simulink model "generic_src"  (Simulink 10.3)
settings: Solver=ode45  StartTime=0.0  StopTime=inf  RelTol=1e-3  EnableMultiTasking=on
undefined symbols (not defined in the file or in its folder): Area_Front, Area_Rear, ay_max_off, ay_max_on, ay_per_mu_max_off, ay_per_mu_max_on, Brake_ratio, brake_valve_ctrl_kP, cat1mode1_higher, cat1mode1_lower, cat1mode2_higher, cat1mode2_lower, cat1mode3_higher, cat1mode3_lower, cat2mode1_higher, cat2mode1_lower, cat2mode2_higher, cat2mode2_lower, cat2mode3_higher, cat2mode3_lower, delta_vel, diff_lock_fac, diff_lock_off, diff_lock_on, ESP_ctrl_kD, ESP_ctrl_kI, ESP_ctrl_kP, ESP_ctrl_restore_kI, ESP_min_throttle_fac, f_ax, f_slip, g, higherlimit_highvel, higherlimit_lowvel, highervel_fac, highervelocity_fac, InitialConditionForIntegrator, limit_acc, limit_selectlow, limit_starting, limit_vdiff, locktime_throttle, lowerlimit_highvel, lowerlimit_lowvel, lowervel_fac, lowervelocity_fac, min_throttle, MPS2KMPH, MSR_ctrl_kD, MSR_ctrl_kI, MSR_ctrl_kP, MSR_min_throttle_fac, PID_kP_sideslip, PID_kP_yawrate, RADpS2RpM, rBrake, RpM2RADpS, SH_SL_switch, sideslip_vel_corr, sidesplip_deviation_max ... (+35)
libraries: CarMaker4SL x136, simulink x55, simulink_extras x6
(part 7 of 9)

== system generic_src/CarMaker/IPG Vehicle/Brake/HydBrakeCU Example/ESP Controller/ESP General System/Signal Handling ==
  ESP In : Inport
  Vehicle Params : Inport  Port=2
  " " : simulink_extras/Transformations/Degrees to Radians
  "  " : simulink_extras/Transformations/Degrees to Radians
  "   " : Gain  Gain=RpM2RADpS
  "     " : Gain  Gain=RpM2RADpS
  "      " : Gain  Gain=RpM2RADpS
  Bus Creator : BusCreator  Inputs=4
  Bus Creator1 : BusCreator  Inputs=4
  Bus Creator2 : BusCreator  Inputs=6
  Bus Creator3 : BusCreator  Inputs=2
  Bus Creator4 : BusCreator  Inputs=2
  Bus Creator5 : BusCreator  Inputs=1
  Bus Creator6 : BusCreator  Inputs=3
  Bus Selector1 : BusSelector  OutputSignals=WheelSpd FL [rpm],WheelSpd FR [rpm],WheelSpd RL [rpm],WheelSpd RR [rpm],Master Cylinder Pressure [bar],Throttle Valve Position,Sensor Longitudinal acceleration [g],Engine Speed [rpm],GearState [-],Torque Converter Speed [rpm],Sensor YawRate [degs],Steering Wheel Angle [deg],Sensor Lateral acceleration [g],Cylinder Pressure FL [bar],Cylinder Pressure FR [bar],Cylinder Pressure RL [bar],Cylinder Pressure RR [bar],Engine crankshaft output torque [Nm],Park Brake Position,Brake Pedal Position
  Bus Selector2 : BusSelector  OutputSignals=SteeringGeometry
  Bus Selector3 : BusSelector  OutputSignals=SteerWheelAng_In,SteerAng_Out
  Gain2 : Gain  Gain=g  SaturateOnIntegerOverflow=on  OutDataTypeStr=Inherit: Same as input  ParamDataTypeStr=Inherit: Same as input
  Gain7 : Gain  Gain=g  SaturateOnIntegerOverflow=on  OutDataTypeStr=Inherit: Same as input  ParamDataTypeStr=Inherit: Same as input
  Lookup Table Dynamic : simulink/Lookup Tables/Lookup Table Dynamic  LookUpMeth=Interpolation-Use End Values  OutDataType=fixdt('double')  OutScaling=[]  OutputDataTypeScalingMode=Specify via dialog  OutDataTypeStr=fixdt('double')  DoSatur=off
  Termiator : Terminator
  Terminator1 : Terminator
  Terminator2 : Terminator
  Terminator4 : Terminator
  rpmin2rad/s : Gain  Gain=RpM2RADpS
  Signal Bus Master Controller : Outport  VectorParamsAs1DForOutWhenUnconnected=off
  Signal Bus ESP : Outport  Port=2  VectorParamsAs1DForOutWhenUnconnected=off
  Signal Bus ASR : Outport  Port=3  VectorParamsAs1DForOutWhenUnconnected=off
  Signal Bus ABS : Outport  Port=4  VectorParamsAs1DForOutWhenUnconnected=off
  Signal Bus HSA : Outport  Port=5  VectorParamsAs1DForOutWhenUnconnected=off
  wires:
  "  "/1 -> Lookup Table Dynamic/1
  rpmin2rad/s/1 -> Bus Creator/1  "WheelSpd_FL"
  Bus Selector1/1 -> rpmin2rad/s/1  "<WheelSpd FL [rpm]>"
  Bus Selector1/2 -> "   "/1  "<WheelSpd FR [rpm]>"
  Bus Selector1/3 -> "     "/1  "<WheelSpd RL [rpm]>"
  Bus Selector1/4 -> "      "/1  "<WheelSpd RR [rpm]>"
  Bus Selector1/7 -> Gain7/1  "<Sensor Longitudinal acceleration [g]>"
  Bus Selector1/5 -> Terminator4/1  "<Master Cylinder Pressure [bar]>"
  Bus Selector1/8 -> Terminator2/1  "<Engine Speed [rpm]>"
  Bus Selector1/9 -> Terminator1/1  "<GearState [-]>"
  Bus Selector1/10 -> Termiator/1  "<Torque Converter Speed [rpm]>"
  Bus Selector1/11 -> " "/1  "<Sensor YawRate [degs]>"
  Bus Selector1/12 -> "  "/1  "<Steering Wheel Angle [deg]>"
  Bus Selector1/13 -> Gain2/1  "<Sensor Lateral acceleration [g]>"
  "   "/1 -> Bus Creator/2  "WheelSpd_FR"
  "     "/1 -> Bus Creator/3  "WheelSpd_RL"
  "      "/1 -> Bus Creator/4  "WheelSpd_RR"
  Gain7/1 -> Bus Creator4/2, Bus Creator2/5  "ax [m/s^2]"
  Bus Selector1/6 -> Bus Creator6/1, Bus Creator2/1, Bus Creator3/2  "<Throttle Valve Position>"
  ESP In/1 -> Bus Selector1/1
  Lookup Table Dynamic/1 -> Bus Creator2/3  "Steer Angle"
  " "/1 -> Bus Creator2/2  "Yaw Rate"
  Gain2/1 -> Bus Creator2/4  "ay [m/s^2]"
  Bus Selector1/15 -> Bus Creator1/2  "<Cylinder Pressure FR [bar]>"
  Bus Selector1/17 -> Bus Creator1/4  "<Cylinder Pressure RR [bar]>"
  Bus Selector1/16 -> Bus Creator1/3  "<Cylinder Pressure RL [bar]>"
  Bus Selector1/14 -> Bus Creator1/1  "<Cylinder Pressure FL [bar]>"
  Bus Creator1/1 -> Bus Creator2/6  "Wheel Cylinder Pressure"
  Bus Creator2/1 -> Signal Bus ESP/1
  Bus Creator/1 -> Bus Creator4/1, Bus Creator3/1  "WheelSpeeds"
  Bus Creator3/1 -> Signal Bus ASR/1
  Bus Selector1/18 -> Bus Creator5/1  "<Engine crankshaft output torque [Nm]>"
  Bus Creator4/1 -> Signal Bus ABS/1
  Bus Creator5/1 -> Signal Bus HSA/1
  Vehicle Params/1 -> Bus Selector2/1
  Bus Selector2/1 -> Bus Selector3/1  "<SteeringGeometry>"
  Bus Selector3/2 -> Lookup Table Dynamic/3  "<SteerAng_Out>"
  Bus Selector3/1 -> Lookup Table Dynamic/2  "<SteerWheelAng_In>"
  Bus Creator6/1 -> Signal Bus Master Controller/1
  Bus Selector1/19 -> Bus Creator6/2  "<Park Brake Position>"
  Bus Selector1/20 -> Bus Creator6/3  "<Brake Pedal Position>"

== system generic_src/CarMaker/IPG Vehicle/PowerTrain/MCU Example/MyMotorCU/Enabled Subsystem/MotMode ==
  Trq_trg : Inport
  rotv : Inport  Port=2
  Compare To Zero : simulink/Logic and Bit Operations/Compare To Zero  relop=<  OutDataTypeStr=uint8  ZeroCross=off
  Compare To Zero1 : simulink/Logic and Bit Operations/Compare To Zero  relop=>=  OutDataTypeStr=uint8  ZeroCross=off
  Gain : Gain  Gain=-1
  Logical Operator : Logic  AllPortsSameDT=off  OutDataTypeStr=boolean
  Logical Operator1 : Logic  AllPortsSameDT=off  OutDataTypeStr=boolean
  Logical Operator2 : Logic  Operator=OR  AllPortsSameDT=off  OutDataTypeStr=boolean
  Relational Operator2 : RelationalOperator  OutDataTypeStr=boolean  RndMeth=Nearest
  Relational Operator3 : RelationalOperator  Operator=<  OutDataTypeStr=boolean  RndMeth=Nearest
  limrotv : Constant  Value=0.5
  Boolean : Outport  VectorParamsAs1DForOutWhenUnconnected=off
  wires:
  Gain/1 -> Relational Operator2/2
  Relational Operator3/1 -> Logical Operator1/2
  limrotv/1 -> Gain/1, Relational Operator3/2
  rotv/1 -> Relational Operator3/1, Relational Operator2/1
  Relational Operator2/1 -> Logical Operator/2
  Compare To Zero/1 -> Logical Operator1/1
  Trq_trg/1 -> Compare To Zero/1, Compare To Zero1/1
  Compare To Zero1/1 -> Logical Operator/1
  Logical Operator1/1 -> Logical Operator2/2
  Logical Operator/1 -> Logical Operator2/1
  Logical Operator2/1 -> Boolean/1

== system generic_src/CarMaker/IPG Vehicle/PowerTrain/MCU Example/MyMotorCU/Enabled Subsystem/if condition ==
  rotv_trg : Inport
  rotv : Inport  Port=2
  lim_rotv : Inport  Port=3
  Abs : Abs
  Compare To Constant : simulink/Logic and Bit Operations/Compare To Constant  relop===  const=-99999  OutDataTypeStr=boolean  ZeroCross=off
  Logical Operator : Logic  AllPortsSameDT=off  OutDataTypeStr=boolean
  Relational Operator : RelationalOperator  Operator=>  OutDataTypeStr=boolean  RndMeth=Nearest
  Boolean : Outport  VectorParamsAs1DForOutWhenUnconnected=off
  wires:
  Abs/1 -> Relational Operator/1
  rotv/1 -> Abs/1
  lim_rotv/1 -> Relational Operator/2
  Relational Operator/1 -> Logical Operator/1
  Compare To Constant/1 -> Logical Operator/2
  rotv_trg/1 -> Compare To Constant/1
  Logical Operator/1 -> Boolean/1

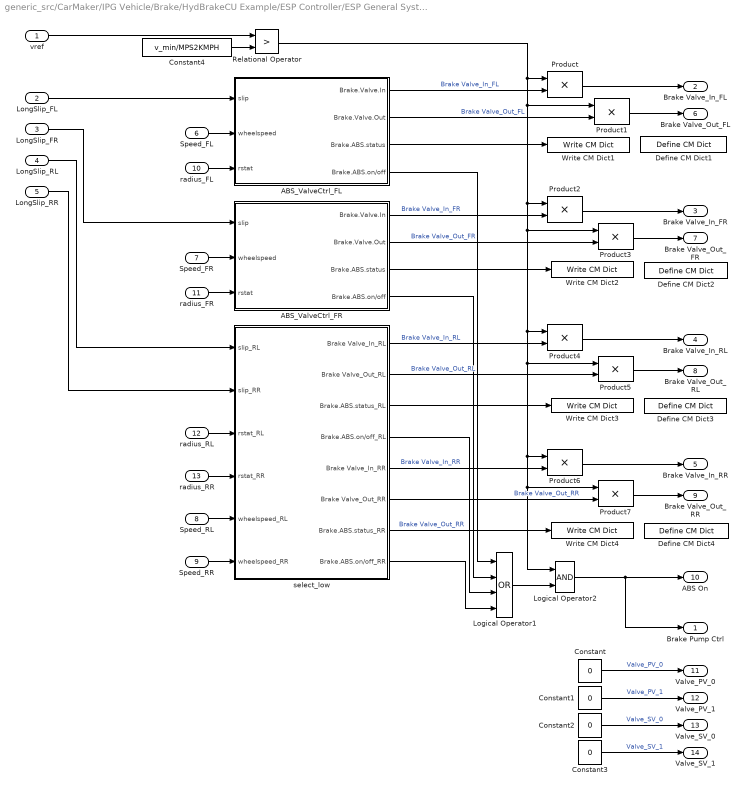
== system generic_src/CarMaker/IPG Vehicle/Brake/HydBrakeCU Example/ESP Controller/ESP General System/ABS/ABS ECU ==
  vref : Inport
  LongSlip_FL : Inport  Port=2
  LongSlip_FR : Inport  Port=3
  LongSlip_RL : Inport  Port=4
  LongSlip_RR : Inport  Port=5
  Speed_FL : Inport  Port=6
  Speed_FR : Inport  Port=7
  Speed_RL : Inport  Port=8
  Speed_RR : Inport  Port=9
  radius_FL : Inport  Port=10
  radius_FR : Inport  Port=11
  radius_RL : Inport  Port=12
  radius_RR : Inport  Port=13
  ABS_ValveCtrl_FL : Subsystem
  ABS_ValveCtrl_FR : Subsystem
  Constant{,1..3} (4 alike) : Constant  Value=0
  Constant4 : Constant  Value=v_min/MPS2KMPH
  Define CM Dict1 : CarMaker4SL/Define CM Dict  xname=ESP.ABS.Status_FL  xmono=off  xtype=Char  xdvaplace=None  xnstates=4  xfirststate=0  xinitial=0
  Define CM Dict2 : CarMaker4SL/Define CM Dict  xname=ESP.ABS.Status_FR  xmono=off  xtype=Char  xdvaplace=None  xnstates=4  xfirststate=0  xinitial=0
  Define CM Dict3 : CarMaker4SL/Define CM Dict  xname=ESP.ABS.Status_RL  xmono=off  xtype=Char  xdvaplace=None  xnstates=4  xfirststate=0  xinitial=0
  Define CM Dict4 : CarMaker4SL/Define CM Dict  xname=ESP.ABS.Status_RR  xmono=off  xtype=Char  xdvaplace=None  xnstates=4  xfirststate=0  xinitial=0
  Logical Operator1 : Logic  Operator=OR  Inputs=4  AllPortsSameDT=off
  Logical Operator2 : Logic  AllPortsSameDT=off
  Product{,1..7} (8 alike) : Product  SaturateOnIntegerOverflow=on  OutDataTypeStr=Inherit: Same as first input
  Relational Operator : RelationalOperator  Operator=>  RndMeth=Nearest
  Write CM Dict1 : CarMaker4SL/Write CM Dict  xname=ESP.ABS.Status_FL  xsync=off
  Write CM Dict2 : CarMaker4SL/Write CM Dict  xname=ESP.ABS.Status_FR  xsync=off
  Write CM Dict3 : CarMaker4SL/Write CM Dict  xname=ESP.ABS.Status_RL  xsync=off
  Write CM Dict4 : CarMaker4SL/Write CM Dict  xname=ESP.ABS.Status_RR  xsync=off
  select_low : Subsystem
  Brake Pump Ctrl : Outport  VectorParamsAs1DForOutWhenUnconnected=off
  Brake Valve_In_FL : Outport  Port=2  VectorParamsAs1DForOutWhenUnconnected=off
  Brake Valve_In_FR : Outport  Port=3  VectorParamsAs1DForOutWhenUnconnected=off
  Brake Valve_In_RL : Outport  Port=4  VectorParamsAs1DForOutWhenUnconnected=off
  Brake Valve_In_RR : Outport  Port=5  VectorParamsAs1DForOutWhenUnconnected=off
  Brake Valve_Out_FL : Outport  Port=6  VectorParamsAs1DForOutWhenUnconnected=off
  Brake Valve_Out_FR : Outport  Port=7  VectorParamsAs1DForOutWhenUnconnected=off
  Brake Valve_Out_RL : Outport  Port=8  VectorParamsAs1DForOutWhenUnconnected=off
  Brake Valve_Out_RR : Outport  Port=9  VectorParamsAs1DForOutWhenUnconnected=off
  ABS On : Outport  Port=10  VectorParamsAs1DForOutWhenUnconnected=off
  Valve_PV_0 : Outport  Port=11  VectorParamsAs1DForOutWhenUnconnected=off
  Valve_PV_1 : Outport  Port=12  VectorParamsAs1DForOutWhenUnconnected=off
  Valve_SV_0 : Outport  Port=13  VectorParamsAs1DForOutWhenUnconnected=off
  Valve_SV_1 : Outport  Port=14  VectorParamsAs1DForOutWhenUnconnected=off
  wires:
  select_low/7(Brake.ABS.status_RR) -> Write CM Dict4/1  "Brake Valve_Out_RR"
  select_low/3(Brake.ABS.status_RL) -> Write CM Dict3/1
  ABS_ValveCtrl_FR/3(Brake.ABS.status) -> Write CM Dict2/1
  ABS_ValveCtrl_FL/4(Brake.ABS.on/off) -> Logical Operator1/1
  ABS_ValveCtrl_FR/4(Brake.ABS.on/off) -> Logical Operator1/2
  select_low/4(Brake.ABS.on/off_RL) -> Logical Operator1/3
  select_low/8(Brake.ABS.on/off_RR) -> Logical Operator1/4
  Constant4/1 -> Relational Operator/2
  Relational Operator/1 -> Product/1, Product6/1, Product7/1, Logical Operator2/1, Product5/1, Product4/1, Product3/1, Product2/1, Product1/1
  ABS_ValveCtrl_FL/1(Brake.Valve.In) -> Product/2  "Brake Valve_In_FL"
  ABS_ValveCtrl_FL/2(Brake.Valve.Out) -> Product1/2  "Brake Valve_Out_FL"
  ABS_ValveCtrl_FR/1(Brake.Valve.In) -> Product2/2  "Brake Valve_In_FR"
  ABS_ValveCtrl_FR/2(Brake.Valve.Out) -> Product3/2  "Brake Valve_Out_FR"
  select_low/1(Brake Valve_In_RL) -> Product4/2  "Brake Valve_In_RL"
  select_low/2(Brake Valve_Out_RL) -> Product5/2  "Brake Valve_Out_RL"
  select_low/5(Brake Valve_In_RR) -> Product6/2  "Brake Valve_In_RR"
  select_low/6(Brake Valve_Out_RR) -> Product7/2  "Brake Valve_Out_RR"
  Product7/1 -> Brake Valve_Out_RR/1
  Product6/1 -> Brake Valve_In_RR/1
  Product5/1 -> Brake Valve_Out_RL/1
  Product4/1 -> Brake Valve_In_RL/1
  Product3/1 -> Brake Valve_Out_FR/1
  Product1/1 -> Brake Valve_Out_FL/1
  LongSlip_FL/1 -> ABS_ValveCtrl_FL/1(slip)
  LongSlip_FR/1 -> ABS_ValveCtrl_FR/1(slip)
  LongSlip_RL/1 -> select_low/1(slip_RL)
  LongSlip_RR/1 -> select_low/2(slip_RR)
  ABS_ValveCtrl_FL/3(Brake.ABS.status) -> Write CM Dict1/1
  Product/1 -> Brake Valve_In_FL/1
  Product2/1 -> Brake Valve_In_FR/1
  Speed_FL/1 -> ABS_ValveCtrl_FL/2(wheelspeed)
  radius_FL/1 -> ABS_ValveCtrl_FL/3(rstat)
  Speed_FR/1 -> ABS_ValveCtrl_FR/2(wheelspeed)
  radius_FR/1 -> ABS_ValveCtrl_FR/3(rstat)
  radius_RL/1 -> select_low/3(rstat_RL)
  radius_RR/1 -> select_low/4(rstat_RR)
  Speed_RL/1 -> select_low/5(wheelspeed_RL)
  Speed_RR/1 -> select_low/6(wheelspeed_RR)
  vref/1 -> Relational Operator/1
  Constant/1 -> Valve_PV_0/1  "Valve_PV_0"
  Constant1/1 -> Valve_PV_1/1  "Valve_PV_1"
  Constant2/1 -> Valve_SV_0/1  "Valve_SV_0"
  Constant3/1 -> Valve_SV_1/1  "Valve_SV_1"
  Logical Operator1/1 -> Logical Operator2/2
  Logical Operator2/1 -> ABS On/1, Brake Pump Ctrl/1

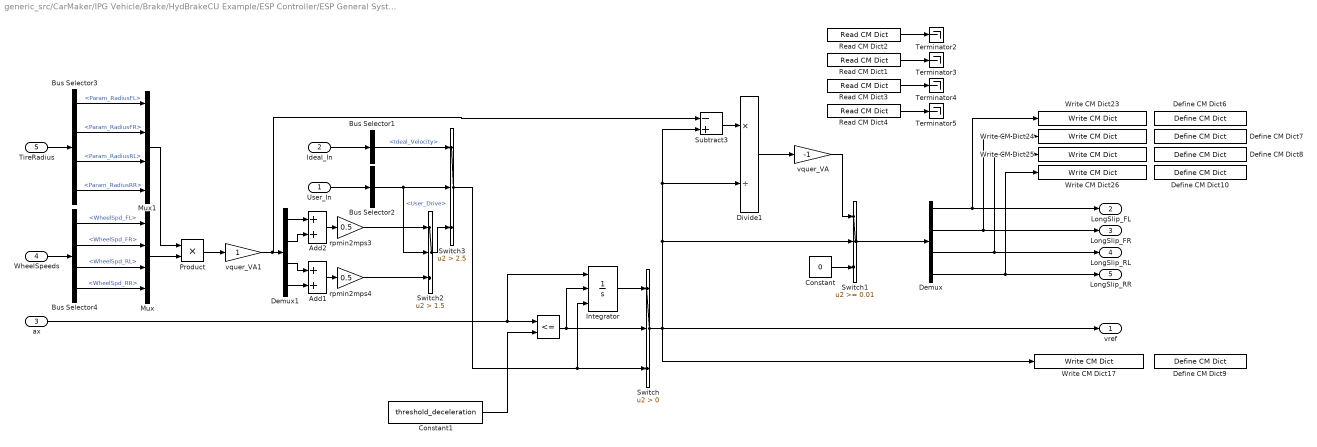
== system generic_src/CarMaker/IPG Vehicle/Brake/HydBrakeCU Example/ESP Controller/ESP General System/ABS/helpsignals estimator ==
  User_In : Inport
  Ideal_In : Inport  Port=2
  ax : Inport  Port=3
  WheelSpeeds : Inport  Port=4
  TireRadius : Inport  Port=5
  " " : RelationalOperator  Operator=<=  OutDataTypeStr=boolean  RndMeth=Nearest
  Add1 : Sum
  Add2 : Sum
  Bus Selector1 : BusSelector  OutputSignals=Ideal_Velocity.Ideal_Velocity
  Bus Selector2 : BusSelector  OutputSignals=User_Drive
  Bus Selector3 : BusSelector  OutputSignals=Param_RadiusFL,Param_RadiusFR,Param_RadiusRL,Param_RadiusRR
  Bus Selector4 : BusSelector  OutputSignals=WheelSpd_FL,WheelSpd_FR,WheelSpd_RL,WheelSpd_RR
  Constant : Constant  Value=0
  Constant1 : Constant  Value=threshold_deceleration
  Define CM Dict10 : CarMaker4SL/Define CM Dict  xname=ESP.ABS.LongSlip_RR  xmono=off  xtype=Double4  xdvaplace=VC  xnstates=0  xfirststate=0  xinitial=0
  Define CM Dict6 : CarMaker4SL/Define CM Dict  xname=ESP.ABS.LongSlip_FL  xmono=off  xtype=Double4  xdvaplace=VC  xnstates=0  xfirststate=0  xinitial=0
  Define CM Dict7 : CarMaker4SL/Define CM Dict  xname=ESP.ABS.LongSlip_FR  xmono=off  xtype=Double4  xdvaplace=VC  xnstates=0  xfirststate=0  xinitial=0
  Define CM Dict8 : CarMaker4SL/Define CM Dict  xname=ESP.ABS.LongSlip_RL  xmono=off  xtype=Double4  xdvaplace=VC  xnstates=0  xfirststate=0  xinitial=0
  Define CM Dict9 : CarMaker4SL/Define CM Dict  xname=ESP.ABS.v_ref  xunit=m/s  xmono=off  xtype=Double4  xdvaplace=VC  xnstates=0  xfirststate=0  xinitial=0
  Demux : Demux
  Demux1 : Demux
  Divide1 : Product  Inputs=*/
  Integrator : Integrator  ExternalReset=rising  InitialConditionSource=external
  Mux : Mux
  Mux1 : Mux
  Product : Product  RndMeth=Zero
  Read CM Dict1 : CarMaker4SL/Read CM Dict  xname=Car.LongSlipFR  xsync=off  xstime=Continuous
  Read CM Dict2 : CarMaker4SL/Read CM Dict  xname=Car.LongSlipFL  xsync=off  xstime=Continuous
  Read CM Dict3 : CarMaker4SL/Read CM Dict  xname=Car.LongSlipRL  xsync=off  xstime=Continuous
  Read CM Dict4 : CarMaker4SL/Read CM Dict  xname=Car.LongSlipRR  xsync=off  xstime=Continuous
  Subtract3 : Sum  Inputs=-+
  Switch : Switch  Criteria=u2 > Threshold
  Switch1 : Switch  Threshold=0.01
  Switch2 : Switch  Criteria=u2 > Threshold  Threshold=1.5
  Switch3 : Switch  Criteria=u2 > Threshold  Threshold=2.5
  Terminator{2..5} (4 alike) : Terminator
  Write CM Dict17 : CarMaker4SL/Write CM Dict  xname=ESP.ABS.v_ref  xsync=off
  Write CM Dict23 : CarMaker4SL/Write CM Dict  xname=ESP.ABS.LongSlip_FL  xsync=off
  Write CM Dict24 : CarMaker4SL/Write CM Dict  xname=ESP.ABS.LongSlip_FR  xsync=off
  Write CM Dict25 : CarMaker4SL/Write CM Dict  xname=ESP.ABS.LongSlip_RL  xsync=off
  Write CM Dict26 : CarMaker4SL/Write CM Dict  xname=ESP.ABS.LongSlip_RR  xsync=off
  rpmin2mps3 : Gain  Gain=0.5
  rpmin2mps4 : Gain  Gain=0.5
  vquer_VA : Gain  Gain=-1
  vquer_VA1 : Gain
  vref : Outport  VectorParamsAs1DForOutWhenUnconnected=off
  LongSlip_FL : Outport  Port=2  VectorParamsAs1DForOutWhenUnconnected=off
  LongSlip_FR : Outport  Port=3  VectorParamsAs1DForOutWhenUnconnected=off
  LongSlip_RL : Outport  Port=4  VectorParamsAs1DForOutWhenUnconnected=off
  LongSlip_RR : Outport  Port=5  VectorParamsAs1DForOutWhenUnconnected=off
  wires:
  Product/1 -> vquer_VA1/1
  Mux1/1 -> Product/1
  Mux/1 -> Product/2
  Subtract3/1 -> Divide1/1
  Divide1/1 -> vquer_VA/1
  vquer_VA/1 -> Switch1/1
  ax/1 -> Integrator/1, " "/1
  Switch3/1 -> Integrator/3, Switch/3
  Demux1/3 -> Add1/1
  Demux1/4 -> Add1/2
  Switch/1 -> Subtract3/2, Divide1/2, Switch1/2, vref/1, Write CM Dict17/1
  Switch1/1 -> Demux/1
  Constant/1 -> Switch1/3
  Demux/1 -> LongSlip_FL/1, Write CM Dict23/1
  Demux/2 -> LongSlip_FR/1, Write CM Dict24/1
  Demux/3 -> LongSlip_RL/1, Write CM Dict25/1
  Demux/4 -> LongSlip_RR/1, Write CM Dict26/1
  vquer_VA1/1 -> Subtract3/1, Demux1/1
  " "/1 -> Integrator/2, Switch/2
  Read CM Dict2/1 -> Terminator2/1
  Read CM Dict1/1 -> Terminator3/1
  Read CM Dict3/1 -> Terminator4/1
  Read CM Dict4/1 -> Terminator5/1
  Demux1/1 -> Add2/1
  Demux1/2 -> Add2/2
  User_In/1 -> Bus Selector2/1
  Add1/1 -> rpmin2mps4/1
  Bus Selector2/1 -> Switch2/2, Switch3/2  "<User_Drive>"
  Add2/1 -> rpmin2mps3/1
  Switch2/1 -> Switch3/3
  Bus Selector1/1 -> Switch3/1  "<Ideal_Velocity>"
  Ideal_In/1 -> Bus Selector1/1
  TireRadius/1 -> Bus Selector3/1
  Bus Selector3/2 -> Mux1/2  "<Param_RadiusFR>"
  Bus Selector3/3 -> Mux1/3  "<Param_RadiusRL>"
  Bus Selector3/4 -> Mux1/4  "<Param_RadiusRR>"
  Bus Selector3/1 -> Mux1/1  "<Param_RadiusFL>"
  WheelSpeeds/1 -> Bus Selector4/1
  Bus Selector4/4 -> Mux/4  "<WheelSpd_RR>"
  Bus Selector4/3 -> Mux/3  "<WheelSpd_RL>"
  Bus Selector4/2 -> Mux/2  "<WheelSpd_FR>"
  Bus Selector4/1 -> Mux/1  "<WheelSpd_FL>"
  rpmin2mps3/1 -> Switch2/1
  rpmin2mps4/1 -> Switch2/3
  Constant1/1 -> " "/2
  Integrator/1 -> Switch/1

== system generic_src/CarMaker/IPG Vehicle/Brake/HydBrakeCU Example/ESP Controller/ESP General System/ASR/BMR ECU ==
  Throttle : Inport
  WheelVelocity [kmph] : Inport  Port=2
  User_In : Inport  Port=3
  Ideal_In : Inport  Port=4
  BMR Controller : Subsystem
  BMR logic : Subsystem
  Bus Creator : BusCreator  Inputs=8
  Bus Creator1 : BusCreator  Inputs=2
  Bus Creator2 : BusCreator  Inputs=2
  Bus Creator3 : BusCreator  Inputs=2
  Differential Lock : Subsystem
  Signal Mapping : Subsystem
  BMR On : Outport  VectorParamsAs1DForOutWhenUnconnected=off
  Brake Valves : Outport  Port=2  VectorParamsAs1DForOutWhenUnconnected=off
  Pilot Valves : Outport  Port=3  VectorParamsAs1DForOutWhenUnconnected=off
  Suctions Valves : Outport  Port=4  VectorParamsAs1DForOutWhenUnconnected=off
  Pump Ctrl : Outport  Port=5  VectorParamsAs1DForOutWhenUnconnected=off
  Diff_Torque : Outport  Port=6  VectorParamsAs1DForOutWhenUnconnected=off
  wires:
  Bus Creator/1 -> Brake Valves/1
  BMR Controller/1(Brake Valve_In_FL) -> Bus Creator/1  "Valve_In_FL"
  BMR Controller/2(Brake Valve_In_FR) -> Bus Creator/2  "Valve_In_FR"
  BMR Controller/3(Brake Valve_In_RL) -> Bus Creator/3  "Valve_In_RL"
  BMR Controller/4(Brake Valve_In_RR) -> Bus Creator/4  "Valve_In_RR"
  BMR Controller/5(Brake Valve_Out_FL) -> Bus Creator/5  "Valve_Out_FL"
  BMR Controller/6(Brake Valve_Out_FR) -> Bus Creator/6  "Valve_Out_FR"
  BMR Controller/7(Brake Valve_Out_RL) -> Bus Creator/7  "Valve_Out_RL"
  BMR Controller/8(Brake Valve_Out_RR) -> Bus Creator/8  "Valve_Out_RR"
  BMR Controller/9(Valve_PV_0) -> Bus Creator2/1  "Valve_PV_0"
  BMR Controller/10(Valve_PV_1) -> Bus Creator2/2  "Valve_PV_1"
  BMR Controller/11(Valve_SV_0) -> Bus Creator1/1  "Valve_SV_0"
  BMR Controller/12(Valve_SV_1) -> Bus Creator1/2  "Valve_SV_1"
  BMR Controller/13(Pump Ctrl) -> Pump Ctrl/1  "PumpCtrl"
  Bus Creator2/1 -> Pilot Valves/1
  Bus Creator1/1 -> Suctions Valves/1
  WheelVelocity [kmph]/1 -> Signal Mapping/2(WheelVelocity)
  Differential Lock/1(FrontDiff_Torque) -> Bus Creator3/1  "FrontDiff_Torque"
  Differential Lock/2(RearDiff_Torque) -> Bus Creator3/2  "RearDiff_Torque"
  Bus Creator3/1 -> Diff_Torque/1
  Ideal_In/1 -> Signal Mapping/3(Ideal_In)
  Signal Mapping/1(v_DrivenL) -> Differential Lock/2(v_DrivenL), BMR logic/1(v_drivenL)
  Signal Mapping/2(v_DrivenR) -> Differential Lock/3(v_DrivenR), BMR logic/2(v_drivenR)
  Signal Mapping/3(v_UndrivenL) -> BMR logic/3(v_undrivenL)
  Signal Mapping/4(v_UndrivenR) -> BMR logic/4(v_undrivenR)
  Throttle/1 -> BMR logic/5(Throttle position)
  BMR logic/1(mode) -> BMR Controller/2(mode)
  BMR logic/2(BMR On) -> BMR Controller/3(BMR On), BMR On/1
  User_In/1 -> BMR Controller/1(User_In), Differential Lock/1(User_In), Signal Mapping/1(User_In)

== system generic_src/CarMaker/IPG Vehicle/Brake/HydBrakeCU Example/ESP Controller/ESP General System/ASR/MSR ECU ==
  Throttle Position : Inport
  WheelVelocity [kmph] : Inport  Port=2
  User_In : Inport  Port=3
  Ideal_In : Inport  Port=4
  MSR logic : Subsystem
  MSR/Gas Controller : Subsystem
  Signal Mapping : Subsystem
  Gas_out : Outport  VectorParamsAs1DForOutWhenUnconnected=off
  MSR On : Outport  Port=2  VectorParamsAs1DForOutWhenUnconnected=off
  wires:
  Throttle Position/1 -> MSR/Gas Controller/1(Throttle_position)
  MSR/Gas Controller/1(MSR_On) -> MSR On/1
  MSR/Gas Controller/2(Gas_Out) -> Gas_out/1
  WheelVelocity [kmph]/1 -> Signal Mapping/1(WheelVelocity)
  User_In/1 -> Signal Mapping/2(User_In)
  Ideal_In/1 -> Signal Mapping/3(Ideal_In)
  Signal Mapping/1(v_DrivenL) -> MSR logic/1(v_drivenL)
  Signal Mapping/2(v_DrivenR) -> MSR logic/2(v_drivenR)
  Signal Mapping/3(v_UndrivenL) -> MSR logic/3(v_undrivenL)
  Signal Mapping/4(v_UndrivenR) -> MSR logic/4(v_undrivenR)
  MSR logic/1(Pseudo_slip) -> MSR/Gas Controller/2(Pseudo_Slip)
  MSR logic/2(reduce torque) -> MSR/Gas Controller/3(close Gas)
  MSR logic/3(hold torque) -> MSR/Gas Controller/4(hold Gas)

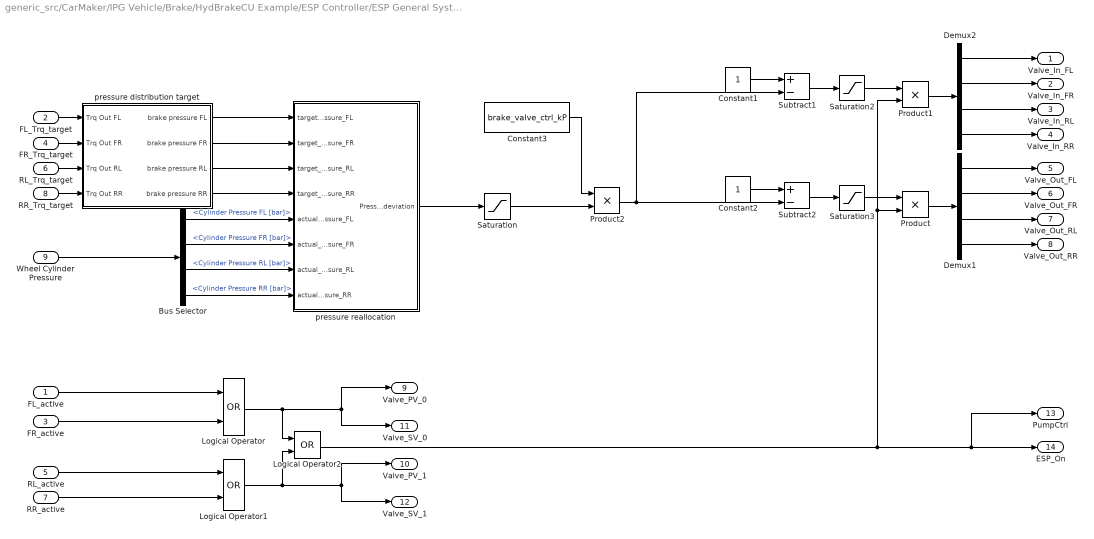
== system generic_src/CarMaker/IPG Vehicle/Brake/HydBrakeCU Example/ESP Controller/ESP General System/ESP/Actuator Brake ==
  FL_active : Inport
  FL_Trq_target : Inport  Port=2
  FR_active : Inport  Port=3
  FR_Trq_target : Inport  Port=4
  RL_active : Inport  Port=5
  RL_Trq_target : Inport  Port=6
  RR_active : Inport  Port=7
  RR_Trq_target : Inport  Port=8
  Wheel Cylinder Pressure : Inport  Port=9
  Bus Selector : BusSelector  OutputSignals=Cylinder Pressure FL [bar],Cylinder Pressure FR [bar],Cylinder Pressure RL [bar],Cylinder Pressure RR [bar]
  Constant1 : Constant
  Constant2 : Constant
  Constant3 : Constant  Value=brake_valve_ctrl_kP
  Demux1 : Demux
  Demux2 : Demux
  Logical Operator : Logic  Operator=OR  AllPortsSameDT=off
  Logical Operator1 : Logic  Operator=OR  AllPortsSameDT=off
  Logical Operator2 : Logic  Operator=OR  AllPortsSameDT=off
  Product : Product  RndMeth=Zero
  Product1 : Product  RndMeth=Zero
  Product2 : Product  RndMeth=Zero
  Saturation : Saturate  UpperLimit=500  LowerLimit=0
  Saturation2 : Saturate  UpperLimit=1  LowerLimit=0
  Saturation3 : Saturate  UpperLimit=1  LowerLimit=0
  Subtract1 : Sum  Inputs=+-
  Subtract2 : Sum  Inputs=+-
  pressure distribution target : Subsystem
  pressure reallocation : Subsystem
  Valve_In_FL : Outport  VectorParamsAs1DForOutWhenUnconnected=off
  Valve_In_FR : Outport  Port=2  VectorParamsAs1DForOutWhenUnconnected=off
  Valve_In_RL : Outport  Port=3  VectorParamsAs1DForOutWhenUnconnected=off
  Valve_In_RR : Outport  Port=4  VectorParamsAs1DForOutWhenUnconnected=off
  Valve_Out_FL : Outport  Port=5  VectorParamsAs1DForOutWhenUnconnected=off
  Valve_Out_FR : Outport  Port=6  VectorParamsAs1DForOutWhenUnconnected=off
  Valve_Out_RL : Outport  Port=7  VectorParamsAs1DForOutWhenUnconnected=off
  Valve_Out_RR : Outport  Port=8  VectorParamsAs1DForOutWhenUnconnected=off
  Valve_PV_0 : Outport  Port=9  VectorParamsAs1DForOutWhenUnconnected=off
  Valve_PV_1 : Outport  Port=10  VectorParamsAs1DForOutWhenUnconnected=off
  Valve_SV_0 : Outport  Port=11  VectorParamsAs1DForOutWhenUnconnected=off
  Valve_SV_1 : Outport  Port=12  VectorParamsAs1DForOutWhenUnconnected=off
  PumpCtrl : Outport  Port=13  VectorParamsAs1DForOutWhenUnconnected=off
  ESP_On : Outport  Port=14  VectorParamsAs1DForOutWhenUnconnected=off
  wires:
  FL_Trq_target/1 -> pressure distribution target/1(Trq Out FL)
  Product2/1 -> Subtract2/2, Subtract1/2
  Saturation/1 -> Product2/2
  Constant1/1 -> Subtract1/1
  Constant2/1 -> Subtract2/1
  FR_Trq_target/1 -> pressure distribution target/2(Trq Out FR)
  FL_active/1 -> Logical Operator/1
  FR_active/1 -> Logical Operator/2
  Logical Operator/1 -> Valve_PV_0/1, Valve_SV_0/1, Logical Operator2/1
  RL_active/1 -> Logical Operator1/1
  RR_active/1 -> Logical Operator1/2
  Logical Operator1/1 -> Valve_PV_1/1, Valve_SV_1/1, Logical Operator2/2
  Logical Operator2/1 -> ESP_On/1, PumpCtrl/1, Product1/2, Product/2
  Subtract1/1 -> Saturation2/1
  Subtract2/1 -> Saturation3/1
  Demux1/1 -> Valve_Out_FL/1
  Demux1/2 -> Valve_Out_FR/1
  RL_Trq_target/1 -> pressure distribution target/3(Trq Out RL)
  RR_Trq_target/1 -> pressure distribution target/4(Trq Out RR)
  Demux1/3 -> Valve_Out_RL/1
  Demux1/4 -> Valve_Out_RR/1
  Demux2/1 -> Valve_In_FL/1
  Demux2/2 -> Valve_In_FR/1
  Demux2/3 -> Valve_In_RL/1
  Demux2/4 -> Valve_In_RR/1
  Saturation3/1 -> Product/1
  Product/1 -> Demux1/1
  Saturation2/1 -> Product1/1
  Product1/1 -> Demux2/1
  Wheel Cylinder Pressure/1 -> Bus Selector/1
  Constant3/1 -> Product2/1
  pressure distribution target/1(brake pressure FL) -> pressure reallocation/1(target_pressure_FL)
  pressure distribution target/2(brake pressure FR) -> pressure reallocation/2(target_pressure_FR)
  pressure distribution target/3(brake pressure RL) -> pressure reallocation/3(target_pressure_RL)
  pressure distribution target/4(brake pressure RR) -> pressure reallocation/4(target_pressure_RR)
  Bus Selector/1 -> pressure reallocation/5(actual_pressure_FL)  "<Cylinder Pressure FL [bar]>"
  Bus Selector/2 -> pressure reallocation/6(actual_pressure_FR)  "<Cylinder Pressure FR [bar]>"
  Bus Selector/3 -> pressure reallocation/7(actual_pressure_RL)  "<Cylinder Pressure RL [bar]>"
  Bus Selector/4 -> pressure reallocation/8(actual_pressure_RR)  "<Cylinder Pressure RR [bar]>"
  pressure reallocation/1(Pressure deviation) -> Saturation/1

== system generic_src/CarMaker/IPG Vehicle/Brake/HydBrakeCU Example/ESP Controller/ESP General System/ESP/ECU ==
  ax : Inport
  Throttle Position : Inport  Port=2
  Yaw Rate : Inport  Port=3
  Steer Angle : Inport  Port=4
  Sideslip : Inport  Port=5
  mu : Inport  Port=6
  ay : Inport  Port=7
  Ideal_In : Inport  Port=8
  Vehicle Params : Inport  Port=9
  User_In : Inport  Port=10
  ECU logic : Subsystem
  Instability detectors : Subsystem
  Motor management strategy : Subsystem
  brake distribution strategy : Subsystem
  Gas_out : Outport  VectorParamsAs1DForOutWhenUnconnected=off
  FL_active : Outport  Port=2  VectorParamsAs1DForOutWhenUnconnected=off
  FL_Trq_target : Outport  Port=3  VectorParamsAs1DForOutWhenUnconnected=off
  FR_active : Outport  Port=4  VectorParamsAs1DForOutWhenUnconnected=off
  FR_Trq_target : Outport  Port=5  VectorParamsAs1DForOutWhenUnconnected=off
  RL_active : Outport  Port=6  VectorParamsAs1DForOutWhenUnconnected=off
  RL_Trq_target : Outport  Port=7  VectorParamsAs1DForOutWhenUnconnected=off
  RR_active : Outport  Port=8  VectorParamsAs1DForOutWhenUnconnected=off
  RR_Trq_target : Outport  Port=9  VectorParamsAs1DForOutWhenUnconnected=off
  wires:
  ECU logic/1(Stabilizing Torque) -> brake distribution strategy/2(Stabilizing Torque)
  Steer Angle/1 -> Instability detectors/1(Steer Angle), brake distribution strategy/1(Steer Angle)
  Yaw Rate/1 -> Instability detectors/2(Yaw Rate)
  brake distribution strategy/1(FL_active) -> FL_active/1
  brake distribution strategy/2(Trq_FL_target) -> FL_Trq_target/1
  brake distribution strategy/3(FR_active) -> FR_active/1
  brake distribution strategy/4(Trq_FR_target) -> FR_Trq_target/1
  brake distribution strategy/5(RL_active) -> RL_active/1
  brake distribution strategy/6(Trq_RL_target) -> RL_Trq_target/1
  brake distribution strategy/7(RR_active) -> RR_active/1
  brake distribution strategy/8(Trq_RR_target) -> RR_Trq_target/1
  Instability detectors/1(SideSlipAngle deviation) -> ECU logic/1(SideSlipAngle deviation)
  Instability detectors/2(YawRate corrected deviation) -> ECU logic/2(YawRate corrected deviation)
  Throttle Position/1 -> Motor management strategy/2(Throttle_position)
  ax/1 -> Motor management strategy/3(ax)
  Motor management strategy/1(Gas_out) -> Gas_out/1
  ay/1 -> Instability detectors/3(ay)
  Instability detectors/3(motormanagement activation) -> Motor management strategy/1(activation DK)
  Sideslip/1 -> Instability detectors/4(Sideslip)
  mu/1 -> ECU logic/3(mu_max), Instability detectors/5(mu_max)
  Ideal_In/1 -> ECU logic/4(Ideal_In), Instability detectors/6(Ideal_In)
  Vehicle Params/1 -> Instability detectors/7(Vehicle Params), brake distribution strategy/3(Vehicle Params)
  User_In/1 -> brake distribution strategy/4(User_In)

== system generic_src/CarMaker/IPG Vehicle/Brake/HydBrakeCU Example/ESP Controller/ESP General System/ESP/helpsignals estimator ==
  Steer Angle : Inport
  Ideal_In : Inport  Port=2
  Vehicle Params : Inport  Port=3
  User_In : Inport  Port=4
  Bus Selector1 : BusSelector  OutputSignals=Ideal_SideSlipAngle
  Bus Selector2 : BusSelector  OutputSignals=User_estimators_on.User_SideSlip_estimator_on,User_estimators_on.User_mue_estimator_on
  Bus Selector3 : BusSelector  OutputSignals=Ideal_mu.Ideal_muFL,Ideal_mu.Ideal_muFR,Ideal_mu.Ideal_muRL,Ideal_mu.Ideal_muRR
  MinMax : MinMax  Inputs=4
  SideSlip estimator : Subsystem
  Switch : Switch  Criteria=u2 > Threshold
  Switch1 : Switch  Criteria=u2 > Threshold
  mue estimator : Subsystem
  SideslipAngle : Outport  VectorParamsAs1DForOutWhenUnconnected=off
  mu : Outport  Port=2  VectorParamsAs1DForOutWhenUnconnected=off
  wires:
  Steer Angle/1 -> SideSlip estimator/1(lenkwinkel)
  mue estimator/1(mue_estimated) -> Switch1/1
  User_In/1 -> Bus Selector2/1
  Bus Selector2/1 -> Switch/2  "<User_SideSlip_estimator_on>"
  Bus Selector1/1 -> Switch/3  "<Ideal_SideSlipAngle>"
  SideSlip estimator/1(SideSlipAngle_estimated) -> Switch/1
  Switch/1 -> SideslipAngle/1
  Bus Selector2/2 -> Switch1/2  "<User_mue_estimator_on>"
  Switch1/1 -> mu/1
  MinMax/1 -> Switch1/3
  Ideal_In/1 -> Bus Selector3/1, mue estimator/1(CarMaker_In), SideSlip estimator/2(CarMaker_In), Bus Selector1/1
  Bus Selector3/3 -> MinMax/3  "<Ideal_muRL>"
  Bus Selector3/2 -> MinMax/2  "<Ideal_muFR>"
  Bus Selector3/4 -> MinMax/4  "<Ideal_muRR>"
  Bus Selector3/1 -> MinMax/1  "<Ideal_muFL>"
  Vehicle Params/1 -> mue estimator/2(Vehicle Params)

== system generic_src/CarMaker/IPG Vehicle/Brake/HydBrakeCU Example/ESP Controller/ESP General System/Master Controller/ABS Off ==
  ABS On : Inport
  ABS Bus : Inport  Port=2
  Bus Creator : BusCreator  Inputs=8
  Bus Creator4 : BusCreator  Inputs='Pilot Valves','Suction Valves','Brake Valves','Pump Ctrl'
  Bus Selector1 : BusSelector  OutputSignals=Valve_In_FL,Valve_In_FR,Valve_In_RL,Valve_In_RR,Valve_Out_FL,Valve_Out_FR,Valve_Out_RL,Valve_Out_RR
  Bus Selector3 : BusSelector  OutputSignals=Pilot Valves,Suction Valves,Brake Valves,Pump Ctrl
  Product{,1..7} (8 alike) : Product  RndMeth=Zero
  ABS Bus Out : Outport  VectorParamsAs1DForOutWhenUnconnected=off
  wires:
  Bus Creator4/1 -> ABS Bus Out/1  "ABS Bus"
  ABS Bus/1 -> Bus Selector3/1
  Bus Selector3/1 -> Bus Creator4/1  "<Pilot Valves>"
  Bus Selector3/2 -> Bus Creator4/2  "<Suction Valves>"
  Bus Selector3/3 -> Bus Selector1/1  "<Brake Valves>"
  Bus Selector3/4 -> Bus Creator4/4  "<Pump Ctrl>"
  Bus Creator/1 -> Bus Creator4/3  "Brake Valves"
  ABS On/1 -> Product7/1, Product6/1, Product5/1, Product4/1, Product3/1, Product2/1, Product1/1, Product/1
  Bus Selector1/1 -> Product/2  "<Valve_In_FL>"
  Product/1 -> Bus Creator/1  "Valve_In_FL"
  Bus Selector1/2 -> Product1/2  "<Valve_In_FR>"
  Product1/1 -> Bus Creator/2  "Valve_In_FR"
  Bus Selector1/3 -> Product2/2  "<Valve_In_RL>"
  Product2/1 -> Bus Creator/3  "Valve_In_RL"
  Bus Selector1/4 -> Product3/2  "<Valve_In_RR>"
  Product3/1 -> Bus Creator/4  "Valve_In_RR"
  Bus Selector1/5 -> Product4/2  "<Valve_Out_FL>"
  Product4/1 -> Bus Creator/5  "Valve_Out_FL"
  Bus Selector1/6 -> Product5/2  "<Valve_Out_FR>"
  Product5/1 -> Bus Creator/6  "Valve_Out_FR"
  Bus Selector1/7 -> Product6/2  "<Valve_Out_RL>"
  Product6/1 -> Bus Creator/7  "Valve_Out_RL"
  Bus Selector1/8 -> Product7/2  "<Valve_Out_RR>"
  Product7/1 -> Bus Creator/8  "Valve_Out_RR"

== system generic_src/CarMaker/IPG Vehicle/Brake/HydBrakeCU Example/ESP Controller/ESP General System/Master Controller/Actuator VC ==
  Signal_In : Inport
  HSA_BrakePark : Inport  Port=2
  Gas_Out_ASR : Inport  Port=3
  Gas_Out_ESP : Inport  Port=4
  HSA_Flag : Inport  Port=5
  ASR_Flag : Inport  Port=6
  ESP_Flag : Inport  Port=7
  Bus Selector3 : BusSelector  OutputSignals=Brake Pedal Position,Park Brake Position
  Bus Creator : BusCreator  Inputs=3
  Constant : Constant
  Constant1 : Constant
  Logical Operator : Logic  Operator=OR  AllPortsSameDT=off  OutDataTypeStr=boolean
  MinMax : MinMax  Inputs=2
  Subtract1 : Sum  Inputs=+-+
  Subtract2 : Sum  Inputs=+-+
  Switch : Switch  Criteria=u2 ~= 0
  Switch1 : Switch  Criteria=u2 ~= 0
  Signals_Out : Outport  VectorParamsAs1DForOutWhenUnconnected=off
  wires:
  Gas_Out_ESP/1 -> Subtract2/3
  Subtract2/1 -> MinMax/1
  ASR_Flag/1 -> Subtract1/2, Logical Operator/2
  Gas_Out_ASR/1 -> Subtract1/3
  Subtract1/1 -> MinMax/2
  Signal_In/1 -> Bus Selector3/1
  Bus Selector3/2 -> Switch/3  "<Park Brake Position>"
  HSA_Flag/1 -> Switch/2
  HSA_BrakePark/1 -> Switch/1
  Bus Creator/1 -> Signals_Out/1
  ESP_Flag/1 -> Subtract2/2, Logical Operator/1
  Switch/1 -> Bus Creator/3  "BrakePark"
  Bus Selector3/1 -> Bus Creator/2  "<Brake Pedal Position>"
  Switch1/1 -> Bus Creator/1  "Load_lim"
  MinMax/1 -> Switch1/1  "Gas"
  Logical Operator/1 -> Switch1/2
  Constant/1 -> Subtract2/1, Subtract1/1
  Constant1/1 -> Switch1/3

== system generic_src/CarMaker/IPG Vehicle/Brake/HydBrakeCU Example/ESP Controller/ESP General System/Master Controller/User Switch ==
  ESP On : Inport
  ASR On : Inport  Port=2
  ABS On : Inport  Port=3
  HSA On : Inport  Port=4
  User In : Inport  Port=5
  Bus Creator6 : BusCreator  Inputs=3
  Bus Selector : BusSelector  OutputSignals=ASR On,MSR On,BMR On
  Bus Selector4 : BusSelector  OutputSignals=User_Switch.User_Switch_Main_off,User_Switch.User_Switch_ESP_off,User_Switch.User_Switch_ASR_off,User_Switch.User_Switch_ABS_off,User_Switch.User_Switch_HSA_off
  Constant : Constant
  Product{,1..9} (10 alike) : Product  RndMeth=Zero
  Subtract{,1..4} (5 alike) : Sum  Inputs=+-
  "ESP On " : Outport  VectorParamsAs1DForOutWhenUnconnected=off
  "ASR On " : Outport  Port=2  VectorParamsAs1DForOutWhenUnconnected=off
  "ABS On " : Outport  Port=3  VectorParamsAs1DForOutWhenUnconnected=off
  "HSA On " : Outport  Port=4  VectorParamsAs1DForOutWhenUnconnected=off
  ASRASR On : Outport  Port=5  VectorParamsAs1DForOutWhenUnconnected=off
  wires:
  ASR On/1 -> Bus Selector/1
  Constant/1 -> Subtract4/1, Subtract3/1, Subtract2/1, Subtract1/1, Subtract/1
  Bus Selector4/1 -> Subtract/2  "<User_Switch_Main_off>"
  Bus Selector4/2 -> Subtract1/2  "<User_Switch_ESP_off>"
  Bus Selector4/3 -> Subtract2/2  "<User_Switch_ASR_off>"
  Bus Selector4/4 -> Subtract3/2  "<User_Switch_ABS_off>"
  Subtract/1 -> Product/1, Product1/1, Product8/1, Product2/1
  Subtract1/1 -> Product/2
  Subtract2/1 -> Product1/2
  Subtract3/1 -> Product2/2
  Product/1 -> Product3/1
  ESP On/1 -> Product3/2
  Product3/1 -> "ESP On "/1  "ESP On"
  Product1/1 -> Product6/1, Product5/1, Product4/1
  Bus Selector/1 -> Product4/2  "<ASR On>"
  Product4/1 -> Bus Creator6/1, ASRASR On/1  "ASR On"
  Bus Selector/2 -> Product5/2  "<MSR On>"
  Product5/1 -> Bus Creator6/2  "MSR On"
  Bus Creator6/1 -> "ASR On "/1  "ASR On"
  Bus Selector/3 -> Product6/2  "<BMR On>"
  Product6/1 -> Bus Creator6/3  "BMR On"
  Product2/1 -> Product7/1
  ABS On/1 -> Product7/2
  Product7/1 -> "ABS On "/1  "ABS On"
  User In/1 -> Bus Selector4/1
  Bus Selector4/5 -> Subtract4/2  "<User_Switch_HSA_off>"
  Subtract4/1 -> Product8/2
  Product8/1 -> Product9/1
  HSA On/1 -> Product9/2
  Product9/1 -> "HSA On "/1  "HSA On"

== system generic_src/CarMaker/IPG Vehicle/Brake/HydBrakeCU Example/ESP Controller/ESP General System/ABS/ABS ECU/ABS_ValveCtrl_FL ==
  note: Control strategy: Trigger criterion S_K
      | S_K combines wheel decceleration control with slip control
      | using weighting factors  K_z and K_\lambda
      | S_K=K_z*z_R + K_\lambda * \lambda_{rel}
      | (see p.127 in M. Burckhardt
      | Fahrwerktechnik:Radschlupfregelsysteme)
  note: Valve Control:
      | Valves are open for a predefined time window.
      | The driving time depends on a trigger criterion (LUT).
      | The treshold change for the valve driving time is
      | continously modified by a repeating sequence.
  note: EITHER ABS is switched on and  S_K is put through
      |  when S_K is becomming bigger the s_{ku}
      | OR output is 0 when S_K is smaller than {sku}_{off}
  slip : Inport
  wheelspeed : Inport  Port=2
  rstat : Inport  Port=3
  Constant : Constant
  Constant1 : Constant  Value=f_slip
  Constant3 : Constant  Value=f_ax
  Derivative : Derivative
  Duty : Subsystem
  Look-Up Table1 : Lookup  InputValues=Valve_LUTin_VA  Table=ValveIn_LUTout_VA  LookUpMeth=Interpolation-Use End Values  SaturateOnIntegerOverflow=on
  Look-Up Table2 : Lookup  InputValues=Valve_LUTin_VA  Table=ValveOut_LUTout_VA  LookUpMeth=Interpolation-Use End Values  SaturateOnIntegerOverflow=on
  Product : Product  SaturateOnIntegerOverflow=on  OutDataTypeStr=Inherit: Same as first input
  Product1 : Product  Inputs=3  InputSameDT=on  SaturateOnIntegerOverflow=on  OutDataTypeStr=Inherit: Same as first input
  Product2 : Product  SaturateOnIntegerOverflow=on  OutDataTypeStr=Inherit: Same as first input
  Rate Transition{1..4} (4 alike) : RateTransition
  Relational Operator : RelationalOperator  Operator=<  SampleTime=0.001  RndMeth=Nearest
  Relational Operator1 : RelationalOperator  Operator=<  SampleTime=0.001  RndMeth=Nearest
  Relay : Relay  OnSwitchValue=sku_VA  OffSwitchValue=sku_off_VA
  Sum : Sum  Inputs=|--  InputSameDT=on  SaturateOnIntegerOverflow=on  OutDataTypeStr=Inherit: Same as first input
  Sum1 : Sum  Inputs=--+  SaturateOnIntegerOverflow=on
  Zero-Order Hold : ZeroOrderHold  SampleTime=t_Sensor
  Brake.Valve.In : Outport  VectorParamsAs1DForOutWhenUnconnected=off
  Brake.Valve.Out : Outport  Port=2  VectorParamsAs1DForOutWhenUnconnected=off
  Brake.ABS.status : Outport  Port=3  VectorParamsAs1DForOutWhenUnconnected=off
  Brake.ABS.on/off : Outport  Port=4  VectorParamsAs1DForOutWhenUnconnected=off
  wires:
  Zero-Order Hold/1 -> Product/1, Relay/1
  Relay/1 -> Rate Transition4/1, Product/2
  Look-Up Table2/1 -> Rate Transition3/1
  Look-Up Table1/1 -> Rate Transition1/1
  Product/1 -> Look-Up Table1/1, Look-Up Table2/1
  Sum/1 -> Zero-Order Hold/1  "S_K"
  Sum1/1 -> Brake.ABS.status/1
  Constant/1 -> Sum1/3
  Relational Operator1/1 -> Brake.Valve.Out/1, Sum1/2
  Relational Operator/1 -> Sum1/1, Brake.Valve.In/1
  Constant3/1 -> Product1/3
  rstat/1 -> Product1/2
  wheelspeed/1 -> Derivative/1
  slip/1 -> Product2/2
  Product1/1 -> Sum/2
  Product2/1 -> Sum/1
  Derivative/1 -> Product1/1
  Constant1/1 -> Product2/1
  Duty/1(SZ) -> Rate Transition2/1
  Rate Transition1/1 -> Relational Operator/2
  Rate Transition3/1 -> Relational Operator1/2
  Rate Transition4/1 -> Brake.ABS.on/off/1
  Rate Transition2/1 -> Relational Operator/1, Relational Operator1/1

== system generic_src/CarMaker/IPG Vehicle/Brake/HydBrakeCU Example/ESP Controller/ESP General System/ABS/ABS ECU/ABS_ValveCtrl_FR ==
  note: Control strategy: Trigger criterion S_K
      | S_K combines wheel decceleration control with slip control
      | using weighting factors  K_z and K_\lambda
      | S_K=K_z*z_R + K_\lambda * \lambda_{rel}
      | (see p.127 in M. Burckhardt
      | Fahrwerktechnik:Radschlupfregelsysteme)
  note: Valve Control:
      | Valves are open for a predefined time window.
      | The driving time depends on a trigger criterion (LUT).
      | The treshold change for the valve driving time is
      | continously modified by a repeating sequence.
  note: EITHER ABS is switched on and  S_K is put through
      |  when S_K is becomming bigger the s_{ku}
      | OR output is 0 when S_K is smaller than {sku}_{off}
  slip : Inport
  wheelspeed : Inport  Port=2
  rstat : Inport  Port=3
  Constant : Constant
  Constant1 : Constant  Value=f_slip
  Constant3 : Constant  Value=f_ax
  Derivative : Derivative
  Duty : Subsystem
  Look-Up Table1 : Lookup  InputValues=Valve_LUTin_VA  Table=ValveIn_LUTout_VA  LookUpMeth=Interpolation-Use End Values  SaturateOnIntegerOverflow=on
  Look-Up Table2 : Lookup  InputValues=Valve_LUTin_VA  Table=ValveOut_LUTout_VA  LookUpMeth=Interpolation-Use End Values  SaturateOnIntegerOverflow=on
  Product : Product  SaturateOnIntegerOverflow=on  OutDataTypeStr=Inherit: Same as first input
  Product1 : Product  Inputs=3  InputSameDT=on  SaturateOnIntegerOverflow=on  OutDataTypeStr=Inherit: Same as first input
  Product2 : Product  SaturateOnIntegerOverflow=on  OutDataTypeStr=Inherit: Same as first input
  Rate Transition{1..4} (4 alike) : RateTransition
  Relational Operator : RelationalOperator  Operator=<  SampleTime=0.001  RndMeth=Nearest
  Relational Operator1 : RelationalOperator  Operator=<  SampleTime=0.001  RndMeth=Nearest
  Relay : Relay  OnSwitchValue=sku_VA  OffSwitchValue=sku_off_VA
  Sum : Sum  Inputs=|--  InputSameDT=on  SaturateOnIntegerOverflow=on  OutDataTypeStr=Inherit: Same as first input
  Sum1 : Sum  Inputs=--+  SaturateOnIntegerOverflow=on
  Zero-Order Hold : ZeroOrderHold  SampleTime=t_Sensor
  Brake.Valve.In : Outport  VectorParamsAs1DForOutWhenUnconnected=off
  Brake.Valve.Out : Outport  Port=2  VectorParamsAs1DForOutWhenUnconnected=off
  Brake.ABS.status : Outport  Port=3  VectorParamsAs1DForOutWhenUnconnected=off
  Brake.ABS.on/off : Outport  Port=4  VectorParamsAs1DForOutWhenUnconnected=off
  wires:
  Zero-Order Hold/1 -> Product/1, Relay/1
  Relay/1 -> Rate Transition4/1, Product/2
  Look-Up Table2/1 -> Rate Transition3/1
  Look-Up Table1/1 -> Rate Transition1/1
  Duty/1(SZ) -> Rate Transition2/1
  Product/1 -> Look-Up Table2/1, Look-Up Table1/1
  Sum/1 -> Zero-Order Hold/1
  Sum1/1 -> Brake.ABS.status/1
  Constant/1 -> Sum1/3
  Relational Operator1/1 -> Sum1/2, Brake.Valve.Out/1
  Relational Operator/1 -> Sum1/1, Brake.Valve.In/1
  Constant3/1 -> Product1/3
  rstat/1 -> Product1/2
  wheelspeed/1 -> Derivative/1
  slip/1 -> Product2/2
  Product1/1 -> Sum/2
  Product2/1 -> Sum/1
  Derivative/1 -> Product1/1
  Constant1/1 -> Product2/1
  Rate Transition2/1 -> Relational Operator/1, Relational Operator1/1
  Rate Transition1/1 -> Relational Operator/2
  Rate Transition3/1 -> Relational Operator1/2
  Rate Transition4/1 -> Brake.ABS.on/off/1

== system generic_src/CarMaker/IPG Vehicle/Brake/HydBrakeCU Example/ESP Controller/ESP General System/ABS/ABS ECU/select_low ==
  note: Control strategy: Trigger criterion S_K
      | S_K combines wheel decceleration control with slip control
      | using weighting factors  K_z and K_\lambda
      | S_K=K_z*z_R + K_\lambda * \lambda_{rel}
      | (see p.127 in M. Burckhardt
      | Fahrwerktechnik:Radschlupfregelsysteme)
  slip_RL : Inport
  slip_RR : Inport  Port=2
  rstat_RL : Inport  Port=3
  rstat_RR : Inport  Port=4
  wheelspeed_RL : Inport  Port=5
  wheelspeed_RR : Inport  Port=6
  ABS_ValveCtrl_rear : Subsystem
  Constant1 : Constant  Value=f_ax
  Constant2 : Constant  Value=f_slip
  Constant3 : Constant  Value=f_ax
  Constant4 : Constant  Value=f_slip
  Derivative : Derivative
  Derivative1 : Derivative
  MinMax : MinMax  Function=max  Inputs=2  InputSameDT=on  SaturateOnIntegerOverflow=on
  Product1 : Product  Inputs=3  InputSameDT=on  SaturateOnIntegerOverflow=on  OutDataTypeStr=Inherit: Same as first input
  Product2 : Product  Inputs=3  InputSameDT=on  SaturateOnIntegerOverflow=on  OutDataTypeStr=Inherit: Same as first input
  Product3 : Product  SaturateOnIntegerOverflow=on  OutDataTypeStr=Inherit: Same as first input
  Product4 : Product  SaturateOnIntegerOverflow=on  OutDataTypeStr=Inherit: Same as first input
  Sum : Sum  Inputs=|--  InputSameDT=on  SaturateOnIntegerOverflow=on  OutDataTypeStr=Inherit: Same as first input
  Sum1 : Sum  Inputs=|--  InputSameDT=on  SaturateOnIntegerOverflow=on  OutDataTypeStr=Inherit: Same as first input
  Brake Valve_In_RL : Outport  VectorParamsAs1DForOutWhenUnconnected=off
  Brake Valve_Out_RL : Outport  Port=2  VectorParamsAs1DForOutWhenUnconnected=off
  Brake.ABS.status_RL : Outport  Port=3  VectorParamsAs1DForOutWhenUnconnected=off
  Brake.ABS.on/off_RL : Outport  Port=4  VectorParamsAs1DForOutWhenUnconnected=off
  Brake Valve_In_RR : Outport  Port=5  VectorParamsAs1DForOutWhenUnconnected=off
  Brake Valve_Out_RR : Outport  Port=6  VectorParamsAs1DForOutWhenUnconnected=off
  Brake.ABS.status_RR : Outport  Port=7  VectorParamsAs1DForOutWhenUnconnected=off
  Brake.ABS.on/off_RR : Outport  Port=8  VectorParamsAs1DForOutWhenUnconnected=off
  wires:
  MinMax/1 -> ABS_ValveCtrl_rear/1(Sk)
  Sum/1 -> MinMax/2
  Sum1/1 -> MinMax/1
  rstat_RL/1 -> Product2/2
  wheelspeed_RL/1 -> Derivative1/1
  slip_RL/1 -> Product3/2
  Constant1/1 -> Product2/3
  Product2/1 -> Sum1/2
  Product3/1 -> Sum1/1
  Derivative1/1 -> Product2/1
  Constant3/1 -> Product1/3
  Product1/1 -> Sum/2
  Product4/1 -> Sum/1
  Derivative/1 -> Product1/1
  ABS_ValveCtrl_rear/1(Brake.Valve.In) -> Brake Valve_In_RR/1, Brake Valve_In_RL/1  "Brake Valve_In_RL"
  ABS_ValveCtrl_rear/2(Brake.Valve.Out) -> Brake Valve_Out_RR/1, Brake Valve_Out_RL/1  "Brake Valve_Out_RL"
  ABS_ValveCtrl_rear/3(Brake.ABS.status) -> Brake.ABS.status_RR/1, Brake.ABS.status_RL/1
  ABS_ValveCtrl_rear/4(Brake.ABS.on/off) -> Brake.ABS.on/off_RR/1, Brake.ABS.on/off_RL/1
  slip_RR/1 -> Product4/2
  wheelspeed_RR/1 -> Derivative/1
  rstat_RR/1 -> Product1/2
  Constant2/1 -> Product3/1
  Constant4/1 -> Product4/1
